simulink library "sm_wheel_loader_lib"  (R2025a)
settings: Solver=VariableStepAuto  StartTime=0.0  StopTime=10.0  RelTol=1e-3
undefined symbols (not defined in the file): AToTOrificeVector, BiPOrificeVector, boomHEArea, boomREArea, BToTOrificeVector, fluids, GRake, GToothL, GToothR, HMPST, HydFcnParams, logLoad, Position, PToAOrificeVector, PToBOrificeVector, RakeL, RakeR, testInput, Wheel_Loader, X, Y, Z
libraries: sm_lib x694, fl_lib x183, nesl_utility x74, SimscapeFluids_lib x62, sdl_lib x25, cvt_components_lib x25, simulink_extras x5, $bdroot x4, wheel_loader_contact_lib x4, ee_lib x2, SignalEditorBlockLib x1, batteryecm_lib x1
(part 15 of 26)

== system sm_wheel_loader_lib/Wheel Loader Vehicle/Actuators/Hydraulic/Valves Linkage/Orifices Lift ==
  Orifice BiP : SimscapeFluids_lib/Isothermal Liquid/Valves & Orifices/Orifices/Orifice (IL)  orifice_type=foundation.enum.constant_variable.variable  constant_orifice_spec=fluids.isothermal_liquid.valves_orifices.orifices.enum.constant_orifice_spec.area  variable_orifice_spec=fluids.isothermal_liquid.valves_orifices.orifices.enum.orifice_spec.table1D_area_opening  orifice_area_constant=1e-3 m^2  p_diff_TLU_constant=[-4, -3, -2, -1, -.5, 0, .5, 1, 2, 3, 4] MPa  vol_flow_TLU_constant=[-2.44, -2.12, -1.68, -1.22, -.84, 0, .85, 1.21, 1.7, 2.09, 2.41] .* 1e-3 m^3/s  S_min=1e-10 m  del_S=0.005 m  open_orientation=fluids.isothermal_liquid.valves_orifices.orifices.enum.orifice_orientation.positive  area_max=0.5e-4 m^2  area_leak=1e-12 m^2  S_TLU=valveData.spoolPosVector mm  orifice_area_TLU=valveData.BiPOrificeAreaVector mm^2  area=inf m^2  Cd=0.7  Re_c=150  smoothing_factor=0  pressure_recovery=simscape.enum.onoff.off  S_vol_flow_TLU=BiPOrificeVector - 1000*(0) mm  p_diff_TLU=[-10000000, -5000000, -2000000, 2000000, 5000000, 10000000] Pa  vol_flow_TLU=[-1e-07, -7.0711e-08, -4.4721e-08, 4.4721e-08, 7.0711e-08, 1e-07; -2.0352e-05, -1.4391e-05, -9.1017e-06, 9.1017e-06, 1.4391e-05, 2.0352e-05; -.0040736, -.0028805, -.0018218, .0018218, .0028805, .0040736; -.011438, -.0080879, -.0051152, .0051152, .0080879, .011438; -.034356, -.024293, -.015364, .015364, .024293, .034356] m^3/s
      settings: InternalSimscapePortConfiguration="{\"Bottom\":[],\"Left\":[{\"id\":\"A\",\"label\":\"A\",\"type\":\"foundation.isothermal_liquid.isothermal_liquid\"},{\"id\":\"S\",\"label\":\"S\",\"type\":\"input\"}],\"Right\":[{\"id\":\"B\",\"label\":\"B\",\"type\":\"foundation.isothermal_liquid.isothermal_liquid\"}],\"Top\":[]}"
  Orifice AT : SimscapeFluids_lib/Isothermal Liquid/Valves & Orifices/Orifices/Orifice (IL)  orifice_type=foundation.enum.constant_variable.variable  constant_orifice_spec=fluids.isothermal_liquid.valves_orifices.orifices.enum.constant_orifice_spec.area  variable_orifice_spec=fluids.isothermal_liquid.valves_orifices.orifices.enum.orifice_spec.table1D_area_opening  orifice_area_constant=1e-3 m^2  p_diff_TLU_constant=[-4, -3, -2, -1, -.5, 0, .5, 1, 2, 3, 4] MPa  vol_flow_TLU_constant=[-2.44, -2.12, -1.68, -1.22, -.84, 0, .85, 1.21, 1.7, 2.09, 2.41] .* 1e-3 m^3/s  S_min=1e-10 m  del_S=0.005 m  open_orientation=fluids.isothermal_liquid.valves_orifices.orifices.enum.orifice_orientation.positive  area_max=0.5e-4 m^2  area_leak=1e-12 m^2  S_TLU=valveData.spoolPosVector mm  orifice_area_TLU=valveData.AtoTOrificeAreaVector mm^2  area=inf m^2  Cd=0.7  Re_c=150  smoothing_factor=0  pressure_recovery=simscape.enum.onoff.off  S_vol_flow_TLU=AToTOrificeVector - 1000*(0) mm  p_diff_TLU=[-10000000, -5000000, -2000000, 2000000, 5000000, 10000000] Pa  vol_flow_TLU=[-1e-07, -7.0711e-08, -4.4721e-08, 4.4721e-08, 7.0711e-08, 1e-07; -2.0352e-05, -1.4391e-05, -9.1017e-06, 9.1017e-06, 1.4391e-05, 2.0352e-05; -.0040736, -.0028805, -.0018218, .0018218, .0028805, .0040736; -.011438, -.0080879, -.0051152, .0051152, .0080879, .011438; -.034356, -.024293, -.015364, .015364, .024293, .034356] m^3/s
      settings: InternalSimscapePortConfiguration="{\"Bottom\":[],\"Left\":[{\"id\":\"A\",\"label\":\"A\",\"type\":\"foundation.isothermal_liquid.isothermal_liquid\"},{\"id\":\"S\",\"label\":\"S\",\"type\":\"input\"}],\"Right\":[{\"id\":\"B\",\"label\":\"B\",\"type\":\"foundation.isothermal_liquid.isothermal_liquid\"}],\"Top\":[]}"
  Orifice BT : SimscapeFluids_lib/Isothermal Liquid/Valves & Orifices/Orifices/Orifice (IL)  orifice_type=foundation.enum.constant_variable.variable  constant_orifice_spec=fluids.isothermal_liquid.valves_orifices.orifices.enum.constant_orifice_spec.area  variable_orifice_spec=fluids.isothermal_liquid.valves_orifices.orifices.enum.orifice_spec.table1D_area_opening  orifice_area_constant=1e-3 m^2  p_diff_TLU_constant=[-4, -3, -2, -1, -.5, 0, .5, 1, 2, 3, 4] MPa  vol_flow_TLU_constant=[-2.44, -2.12, -1.68, -1.22, -.84, 0, .85, 1.21, 1.7, 2.09, 2.41] .* 1e-3 m^3/s  S_min=1e-10 m  del_S=0.005 m  open_orientation=fluids.isothermal_liquid.valves_orifices.orifices.enum.orifice_orientation.positive  area_max=0.5e-4 m^2  area_leak=1e-12 m^2  S_TLU=valveData.spoolPosVector mm  orifice_area_TLU=valveData.BtoTOrificeAreaVector mm^2  area=inf m^2  Cd=0.7  Re_c=150  smoothing_factor=0  pressure_recovery=simscape.enum.onoff.off  S_vol_flow_TLU=BToTOrificeVector - 1000*(0) mm  p_diff_TLU=[-10000000, -5000000, -2000000, 2000000, 5000000, 10000000] Pa  vol_flow_TLU=[-1e-07, -7.0711e-08, -4.4721e-08, 4.4721e-08, 7.0711e-08, 1e-07; -2.0352e-05, -1.4391e-05, -9.1017e-06, 9.1017e-06, 1.4391e-05, 2.0352e-05; -.0040736, -.0028805, -.0018218, .0018218, .0028805, .0040736; -.011438, -.0080879, -.0051152, .0051152, .0080879, .011438; -.034356, -.024293, -.015364, .015364, .024293, .034356] m^3/s
      settings: InternalSimscapePortConfiguration="{\"Bottom\":[],\"Left\":[{\"id\":\"A\",\"label\":\"A\",\"type\":\"foundation.isothermal_liquid.isothermal_liquid\"},{\"id\":\"S\",\"label\":\"S\",\"type\":\"input\"}],\"Right\":[{\"id\":\"B\",\"label\":\"B\",\"type\":\"foundation.isothermal_liquid.isothermal_liquid\"}],\"Top\":[]}"
  Orifice PA : SimscapeFluids_lib/Isothermal Liquid/Valves & Orifices/Orifices/Orifice (IL)  orifice_type=foundation.enum.constant_variable.variable  constant_orifice_spec=fluids.isothermal_liquid.valves_orifices.orifices.enum.constant_orifice_spec.area  variable_orifice_spec=fluids.isothermal_liquid.valves_orifices.orifices.enum.orifice_spec.table1D_area_opening  orifice_area_constant=1e-3 m^2  p_diff_TLU_constant=[-4, -3, -2, -1, -.5, 0, .5, 1, 2, 3, 4] MPa  vol_flow_TLU_constant=[-2.44, -2.12, -1.68, -1.22, -.84, 0, .85, 1.21, 1.7, 2.09, 2.41] .* 1e-3 m^3/s  S_min=1e-10 m  del_S=0.005 m  open_orientation=fluids.isothermal_liquid.valves_orifices.orifices.enum.orifice_orientation.positive  area_max=0.5e-4 m^2  area_leak=1e-12 m^2  S_TLU=valveData.spoolPosVector mm  orifice_area_TLU=valveData.PtoAOrificeAreaVector mm^2  area=inf m^2  Cd=0.7  Re_c=150  smoothing_factor=0  pressure_recovery=simscape.enum.onoff.off  S_vol_flow_TLU=PToAOrificeVector - 1000*(0) mm  p_diff_TLU=[-10000000, -5000000, -2000000, 2000000, 5000000, 10000000] Pa  vol_flow_TLU=[-1e-07, -7.0711e-08, -4.4721e-08, 4.4721e-08, 7.0711e-08, 1e-07; -2.0352e-05, -1.4391e-05, -9.1017e-06, 9.1017e-06, 1.4391e-05, 2.0352e-05; -.0040736, -.0028805, -.0018218, .0018218, .0028805, .0040736; -.011438, -.0080879, -.0051152, .0051152, .0080879, .011438; -.034356, -.024293, -.015364, .015364, .024293, .034356] m^3/s
      settings: InternalSimscapePortConfiguration="{\"Bottom\":[],\"Left\":[{\"id\":\"A\",\"label\":\"A\",\"type\":\"foundation.isothermal_liquid.isothermal_liquid\"},{\"id\":\"S\",\"label\":\"S\",\"type\":\"input\"}],\"Right\":[{\"id\":\"B\",\"label\":\"B\",\"type\":\"foundation.isothermal_liquid.isothermal_liquid\"}],\"Top\":[]}"
  Orifice PB : SimscapeFluids_lib/Isothermal Liquid/Valves & Orifices/Orifices/Orifice (IL)  orifice_type=foundation.enum.constant_variable.variable  constant_orifice_spec=fluids.isothermal_liquid.valves_orifices.orifices.enum.constant_orifice_spec.area  variable_orifice_spec=fluids.isothermal_liquid.valves_orifices.orifices.enum.orifice_spec.table1D_area_opening  orifice_area_constant=1e-3 m^2  p_diff_TLU_constant=[-4, -3, -2, -1, -.5, 0, .5, 1, 2, 3, 4] MPa  vol_flow_TLU_constant=[-2.44, -2.12, -1.68, -1.22, -.84, 0, .85, 1.21, 1.7, 2.09, 2.41] .* 1e-3 m^3/s  S_min=1e-10 m  del_S=0.005 m  open_orientation=fluids.isothermal_liquid.valves_orifices.orifices.enum.orifice_orientation.positive  area_max=0.5e-4 m^2  area_leak=1e-12 m^2  S_TLU=valveData.spoolPosVector mm  orifice_area_TLU=valveData.PtoBOrificeAreaVector mm^2  area=inf m^2  Cd=0.7  Re_c=150  smoothing_factor=0  pressure_recovery=simscape.enum.onoff.off  S_vol_flow_TLU=PToBOrificeVector - 1000*(0) mm  p_diff_TLU=[-10000000, -5000000, -2000000, 2000000, 5000000, 10000000] Pa  vol_flow_TLU=[-1e-07, -7.0711e-08, -4.4721e-08, 4.4721e-08, 7.0711e-08, 1e-07; -2.0352e-05, -1.4391e-05, -9.1017e-06, 9.1017e-06, 1.4391e-05, 2.0352e-05; -.0040736, -.0028805, -.0018218, .0018218, .0028805, .0040736; -.011438, -.0080879, -.0051152, .0051152, .0080879, .011438; -.034356, -.024293, -.015364, .015364, .024293, .034356] m^3/s
      settings: InternalSimscapePortConfiguration="{\"Bottom\":[],\"Left\":[{\"id\":\"A\",\"label\":\"A\",\"type\":\"foundation.isothermal_liquid.isothermal_liquid\"},{\"id\":\"S\",\"label\":\"S\",\"type\":\"input\"}],\"Right\":[{\"id\":\"B\",\"label\":\"B\",\"type\":\"foundation.isothermal_liquid.isothermal_liquid\"}],\"Top\":[]}"
  PS Abs : fl_lib/Physical Signals/Nonlinear Operators/PS Abs  ZeroCross=true
      settings: InternalSimscapePortConfiguration="{\"Bottom\":[],\"Left\":[{\"id\":\"I\",\"label\":\"\",\"type\":\"input\"}],\"Right\":[{\"id\":\"O\",\"label\":\"\",\"type\":\"output\"}],\"Top\":[]}"
  PS Gain : fl_lib/Physical Signals/Functions/PS Gain  gain=-1
  PS Gain1 : fl_lib/Physical Signals/Functions/PS Gain  gain=-1
  S : PMIOPort  Side=Left
  P : PMIOPort  Port=2  Side=Left
  T : PMIOPort  Port=3  Side=Left
  BiPIn : PMIOPort  Port=4  Side=Left
  A : PMIOPort  Port=5  Side=Right
  B : PMIOPort  Port=6  Side=Right
  BiPOut : PMIOPort  Port=7  Side=Right
  connections:
  Orifice BT/LConn2 -- PS Gain1/RConn1
  Orifice PA/LConn2 -- PS Gain/RConn1
  PS Gain1/LConn1 -- Orifice AT/LConn2 -- S/RConn1 -- PS Abs/LConn1 -- Orifice PB/LConn2 -- PS Gain/LConn1
  Orifice BT/RConn1 -- Orifice AT/RConn1 -- T/RConn1
  Orifice BiP/RConn1 -- BiPOut/RConn1
  Orifice BiP/LConn1 -- BiPIn/RConn1
  Orifice PA/RConn1 -- A/RConn1 -- Orifice AT/LConn1
  Orifice PA/LConn1 -- P/RConn1 -- Orifice PB/LConn1
  Orifice PB/RConn1 -- B/RConn1 -- Orifice BT/LConn1
  PS Abs/RConn1 -- Orifice BiP/LConn2

== system sm_wheel_loader_lib/Wheel Loader Vehicle/Actuators/Hydraulic/Valves Linkage/Orifices Tilt ==
  Orifice BiP : SimscapeFluids_lib/Isothermal Liquid/Valves & Orifices/Orifices/Orifice (IL)  orifice_type=foundation.enum.constant_variable.variable  constant_orifice_spec=fluids.isothermal_liquid.valves_orifices.orifices.enum.constant_orifice_spec.area  variable_orifice_spec=fluids.isothermal_liquid.valves_orifices.orifices.enum.orifice_spec.table1D_area_opening  orifice_area_constant=1e-3 m^2  p_diff_TLU_constant=[-4, -3, -2, -1, -.5, 0, .5, 1, 2, 3, 4] MPa  vol_flow_TLU_constant=[-2.44, -2.12, -1.68, -1.22, -.84, 0, .85, 1.21, 1.7, 2.09, 2.41] .* 1e-3 m^3/s  S_min=1e-10 m  del_S=0.005 m  open_orientation=fluids.isothermal_liquid.valves_orifices.orifices.enum.orifice_orientation.positive  area_max=0.5e-4 m^2  area_leak=1e-12 m^2  S_TLU=valveData.spoolPosVector mm  orifice_area_TLU=valveData.BiPOrificeAreaVector mm^2  area=inf m^2  Cd=0.7  Re_c=150  smoothing_factor=0  pressure_recovery=simscape.enum.onoff.off  S_vol_flow_TLU=BiPOrificeVector - 1000*(0) mm  p_diff_TLU=[-10000000, -5000000, -2000000, 2000000, 5000000, 10000000] Pa  vol_flow_TLU=[-1e-07, -7.0711e-08, -4.4721e-08, 4.4721e-08, 7.0711e-08, 1e-07; -2.0352e-05, -1.4391e-05, -9.1017e-06, 9.1017e-06, 1.4391e-05, 2.0352e-05; -.0040736, -.0028805, -.0018218, .0018218, .0028805, .0040736; -.011438, -.0080879, -.0051152, .0051152, .0080879, .011438; -.034356, -.024293, -.015364, .015364, .024293, .034356] m^3/s
      settings: InternalSimscapePortConfiguration="{\"Bottom\":[],\"Left\":[{\"id\":\"A\",\"label\":\"A\",\"type\":\"foundation.isothermal_liquid.isothermal_liquid\"},{\"id\":\"S\",\"label\":\"S\",\"type\":\"input\"}],\"Right\":[{\"id\":\"B\",\"label\":\"B\",\"type\":\"foundation.isothermal_liquid.isothermal_liquid\"}],\"Top\":[]}"
  Orifice AT : SimscapeFluids_lib/Isothermal Liquid/Valves & Orifices/Orifices/Orifice (IL)  orifice_type=foundation.enum.constant_variable.variable  constant_orifice_spec=fluids.isothermal_liquid.valves_orifices.orifices.enum.constant_orifice_spec.area  variable_orifice_spec=fluids.isothermal_liquid.valves_orifices.orifices.enum.orifice_spec.table1D_area_opening  orifice_area_constant=1e-3 m^2  p_diff_TLU_constant=[-4, -3, -2, -1, -.5, 0, .5, 1, 2, 3, 4] MPa  vol_flow_TLU_constant=[-2.44, -2.12, -1.68, -1.22, -.84, 0, .85, 1.21, 1.7, 2.09, 2.41] .* 1e-3 m^3/s  S_min=1e-10 m  del_S=0.005 m  open_orientation=fluids.isothermal_liquid.valves_orifices.orifices.enum.orifice_orientation.positive  area_max=0.5e-4 m^2  area_leak=1e-12 m^2  S_TLU=valveData.spoolPosVector mm  orifice_area_TLU=valveData.AtoTOrificeAreaVector mm^2  area=inf m^2  Cd=0.7  Re_c=150  smoothing_factor=0  pressure_recovery=simscape.enum.onoff.off  S_vol_flow_TLU=AToTOrificeVector - 1000*(0) mm  p_diff_TLU=[-10000000, -5000000, -2000000, 2000000, 5000000, 10000000] Pa  vol_flow_TLU=[-1e-07, -7.0711e-08, -4.4721e-08, 4.4721e-08, 7.0711e-08, 1e-07; -2.0352e-05, -1.4391e-05, -9.1017e-06, 9.1017e-06, 1.4391e-05, 2.0352e-05; -.0040736, -.0028805, -.0018218, .0018218, .0028805, .0040736; -.011438, -.0080879, -.0051152, .0051152, .0080879, .011438; -.034356, -.024293, -.015364, .015364, .024293, .034356] m^3/s
      settings: InternalSimscapePortConfiguration="{\"Bottom\":[],\"Left\":[{\"id\":\"A\",\"label\":\"A\",\"type\":\"foundation.isothermal_liquid.isothermal_liquid\"},{\"id\":\"S\",\"label\":\"S\",\"type\":\"input\"}],\"Right\":[{\"id\":\"B\",\"label\":\"B\",\"type\":\"foundation.isothermal_liquid.isothermal_liquid\"}],\"Top\":[]}"
  Orifice BT : SimscapeFluids_lib/Isothermal Liquid/Valves & Orifices/Orifices/Orifice (IL)  orifice_type=foundation.enum.constant_variable.variable  constant_orifice_spec=fluids.isothermal_liquid.valves_orifices.orifices.enum.constant_orifice_spec.area  variable_orifice_spec=fluids.isothermal_liquid.valves_orifices.orifices.enum.orifice_spec.table1D_area_opening  orifice_area_constant=1e-3 m^2  p_diff_TLU_constant=[-4, -3, -2, -1, -.5, 0, .5, 1, 2, 3, 4] MPa  vol_flow_TLU_constant=[-2.44, -2.12, -1.68, -1.22, -.84, 0, .85, 1.21, 1.7, 2.09, 2.41] .* 1e-3 m^3/s  S_min=1e-10 m  del_S=0.005 m  open_orientation=fluids.isothermal_liquid.valves_orifices.orifices.enum.orifice_orientation.positive  area_max=0.5e-4 m^2  area_leak=1e-12 m^2  S_TLU=valveData.spoolPosVector mm  orifice_area_TLU=valveData.BtoTOrificeAreaVector mm^2  area=inf m^2  Cd=0.7  Re_c=150  smoothing_factor=0  pressure_recovery=simscape.enum.onoff.off  S_vol_flow_TLU=BToTOrificeVector - 1000*(0) mm  p_diff_TLU=[-10000000, -5000000, -2000000, 2000000, 5000000, 10000000] Pa  vol_flow_TLU=[-1e-07, -7.0711e-08, -4.4721e-08, 4.4721e-08, 7.0711e-08, 1e-07; -2.0352e-05, -1.4391e-05, -9.1017e-06, 9.1017e-06, 1.4391e-05, 2.0352e-05; -.0040736, -.0028805, -.0018218, .0018218, .0028805, .0040736; -.011438, -.0080879, -.0051152, .0051152, .0080879, .011438; -.034356, -.024293, -.015364, .015364, .024293, .034356] m^3/s
      settings: InternalSimscapePortConfiguration="{\"Bottom\":[],\"Left\":[{\"id\":\"A\",\"label\":\"A\",\"type\":\"foundation.isothermal_liquid.isothermal_liquid\"},{\"id\":\"S\",\"label\":\"S\",\"type\":\"input\"}],\"Right\":[{\"id\":\"B\",\"label\":\"B\",\"type\":\"foundation.isothermal_liquid.isothermal_liquid\"}],\"Top\":[]}"
  Orifice PA : SimscapeFluids_lib/Isothermal Liquid/Valves & Orifices/Orifices/Orifice (IL)  orifice_type=foundation.enum.constant_variable.variable  constant_orifice_spec=fluids.isothermal_liquid.valves_orifices.orifices.enum.constant_orifice_spec.area  variable_orifice_spec=fluids.isothermal_liquid.valves_orifices.orifices.enum.orifice_spec.table1D_area_opening  orifice_area_constant=1e-3 m^2  p_diff_TLU_constant=[-4, -3, -2, -1, -.5, 0, .5, 1, 2, 3, 4] MPa  vol_flow_TLU_constant=[-2.44, -2.12, -1.68, -1.22, -.84, 0, .85, 1.21, 1.7, 2.09, 2.41] .* 1e-3 m^3/s  S_min=1e-10 m  del_S=0.005 m  open_orientation=fluids.isothermal_liquid.valves_orifices.orifices.enum.orifice_orientation.positive  area_max=0.5e-4 m^2  area_leak=1e-12 m^2  S_TLU=valveData.spoolPosVector mm  orifice_area_TLU=valveData.PtoAOrificeAreaVector mm^2  area=inf m^2  Cd=0.7  Re_c=150  smoothing_factor=0  pressure_recovery=simscape.enum.onoff.off  S_vol_flow_TLU=PToAOrificeVector - 1000*(0) mm  p_diff_TLU=[-10000000, -5000000, -2000000, 2000000, 5000000, 10000000] Pa  vol_flow_TLU=[-1e-07, -7.0711e-08, -4.4721e-08, 4.4721e-08, 7.0711e-08, 1e-07; -2.0352e-05, -1.4391e-05, -9.1017e-06, 9.1017e-06, 1.4391e-05, 2.0352e-05; -.0040736, -.0028805, -.0018218, .0018218, .0028805, .0040736; -.011438, -.0080879, -.0051152, .0051152, .0080879, .011438; -.034356, -.024293, -.015364, .015364, .024293, .034356] m^3/s
      settings: InternalSimscapePortConfiguration="{\"Bottom\":[],\"Left\":[{\"id\":\"A\",\"label\":\"A\",\"type\":\"foundation.isothermal_liquid.isothermal_liquid\"},{\"id\":\"S\",\"label\":\"S\",\"type\":\"input\"}],\"Right\":[{\"id\":\"B\",\"label\":\"B\",\"type\":\"foundation.isothermal_liquid.isothermal_liquid\"}],\"Top\":[]}"
  Orifice PB : SimscapeFluids_lib/Isothermal Liquid/Valves & Orifices/Orifices/Orifice (IL)  orifice_type=foundation.enum.constant_variable.variable  constant_orifice_spec=fluids.isothermal_liquid.valves_orifices.orifices.enum.constant_orifice_spec.area  variable_orifice_spec=fluids.isothermal_liquid.valves_orifices.orifices.enum.orifice_spec.table1D_area_opening  orifice_area_constant=1e-3 m^2  p_diff_TLU_constant=[-4, -3, -2, -1, -.5, 0, .5, 1, 2, 3, 4] MPa  vol_flow_TLU_constant=[-2.44, -2.12, -1.68, -1.22, -.84, 0, .85, 1.21, 1.7, 2.09, 2.41] .* 1e-3 m^3/s  S_min=1e-10 m  del_S=0.005 m  open_orientation=fluids.isothermal_liquid.valves_orifices.orifices.enum.orifice_orientation.positive  area_max=0.5e-4 m^2  area_leak=1e-12 m^2  S_TLU=valveData.spoolPosVector mm  orifice_area_TLU=valveData.PtoBOrificeAreaVector mm^2  area=inf m^2  Cd=0.7  Re_c=150  smoothing_factor=0  pressure_recovery=simscape.enum.onoff.off  S_vol_flow_TLU=PToBOrificeVector - 1000*(0) mm  p_diff_TLU=[-10000000, -5000000, -2000000, 2000000, 5000000, 10000000] Pa  vol_flow_TLU=[-1e-07, -7.0711e-08, -4.4721e-08, 4.4721e-08, 7.0711e-08, 1e-07; -2.0352e-05, -1.4391e-05, -9.1017e-06, 9.1017e-06, 1.4391e-05, 2.0352e-05; -.0040736, -.0028805, -.0018218, .0018218, .0028805, .0040736; -.011438, -.0080879, -.0051152, .0051152, .0080879, .011438; -.034356, -.024293, -.015364, .015364, .024293, .034356] m^3/s
      settings: InternalSimscapePortConfiguration="{\"Bottom\":[],\"Left\":[{\"id\":\"A\",\"label\":\"A\",\"type\":\"foundation.isothermal_liquid.isothermal_liquid\"},{\"id\":\"S\",\"label\":\"S\",\"type\":\"input\"}],\"Right\":[{\"id\":\"B\",\"label\":\"B\",\"type\":\"foundation.isothermal_liquid.isothermal_liquid\"}],\"Top\":[]}"
  PS Abs : fl_lib/Physical Signals/Nonlinear Operators/PS Abs  ZeroCross=true
      settings: InternalSimscapePortConfiguration="{\"Bottom\":[],\"Left\":[{\"id\":\"I\",\"label\":\"\",\"type\":\"input\"}],\"Right\":[{\"id\":\"O\",\"label\":\"\",\"type\":\"output\"}],\"Top\":[]}"
  PS Gain : fl_lib/Physical Signals/Functions/PS Gain  gain=-1
  PS Gain1 : fl_lib/Physical Signals/Functions/PS Gain  gain=-1
  S : PMIOPort  Side=Left
  P : PMIOPort  Port=2  Side=Left
  T : PMIOPort  Port=3  Side=Left
  BiPIn : PMIOPort  Port=4  Side=Left
  A : PMIOPort  Port=5  Side=Right
  B : PMIOPort  Port=6  Side=Right
  BiPOut : PMIOPort  Port=7  Side=Right
  connections:
  Orifice BT/LConn2 -- PS Gain1/RConn1
  Orifice PA/LConn2 -- PS Gain/RConn1
  PS Abs/LConn1 -- S/RConn1 -- PS Gain/LConn1 -- Orifice PB/LConn2 -- Orifice AT/LConn2 -- PS Gain1/LConn1
  T/RConn1 -- Orifice AT/RConn1 -- Orifice BT/RConn1
  Orifice BiP/RConn1 -- BiPOut/RConn1
  Orifice BiP/LConn1 -- BiPIn/RConn1
  Orifice PA/RConn1 -- A/RConn1 -- Orifice AT/LConn1
  Orifice PA/LConn1 -- P/RConn1 -- Orifice PB/LConn1
  Orifice BT/LConn1 -- Orifice PB/RConn1 -- B/RConn1
  PS Abs/RConn1 -- Orifice BiP/LConn2

== system sm_wheel_loader_lib/Wheel Loader Vehicle/Actuators/Ideal/Power Draw/Limit w ==
  PS Abs : fl_lib/Physical Signals/Nonlinear Operators/PS Abs  ZeroCross=true
      settings: InternalSimscapePortConfiguration="{\"Bottom\":[],\"Left\":[{\"id\":\"I\",\"label\":\"\",\"type\":\"input\"}],\"Right\":[{\"id\":\"O\",\"label\":\"\",\"type\":\"output\"}],\"Top\":[]}"
  PS Constant : fl_lib/Physical Signals/Sources/PS Constant  constant=1e-3 rad/s
  PS Max : fl_lib/Physical Signals/Nonlinear Operators/PS Max  ZeroCross=true
      settings: InternalSimscapePortConfiguration="{\"Bottom\":[],\"Left\":[{\"id\":\"I1\",\"label\":\"\",\"type\":\"input\"},{\"id\":\"I2\",\"label\":\"\",\"type\":\"input\"}],\"Right\":[{\"id\":\"O\",\"label\":\"\",\"type\":\"output\"}],\"Top\":[]}"
  PS Product : fl_lib/Physical Signals/Functions/PS Product
  PS Sign : fl_lib/Physical Signals/Nonlinear Operators/PS Sign
      settings: InternalSimscapePortConfiguration="{\"Bottom\":[],\"Left\":[{\"id\":\"I\",\"label\":\"\",\"type\":\"input\"}],\"Right\":[{\"id\":\"O\",\"label\":\"\",\"type\":\"output\"}],\"Top\":[]}"
  wLim : PMIOPort  Side=Right
  w : PMIOPort  Port=2  Side=Left
  connections:
  wLim/RConn1 -- PS Product/RConn1
  PS Max/LConn1 -- PS Abs/RConn1
  PS Max/LConn2 -- PS Constant/RConn1
  PS Product/LConn2 -- PS Max/RConn1
  w/RConn1 -- PS Sign/LConn1 -- PS Abs/LConn1
  PS Product/LConn1 -- PS Sign/RConn1

== system sm_wheel_loader_lib/Wheel Loader Vehicle/Driveline/Driveline/Driveline 1D/Driveline ==
  Damper : fl_lib/Mechanical/Rotational Elements/Rotational Damper  D=HMPST.DriveshaftF.D N*m*s/rad  w_specify=off  w_priority=None  w=0 rad/s  w_nominal_specify=off  w_nominal_value=1  w_nominal_unit=rad/s  t_specify=off  t_priority=None  t=0 N*m  t_nominal_specify=off  t_nominal_value=1  t_nominal_unit=N*m
  Differential Front : sdl_lib/Gears/Differential  driveshaft_location=2  cd_ratio=HMPST.Differential.Ratio  friction_model=2  efficiency=[ 0.99 0.99 ]  temperature_TLU=[ 280 300 320 ] K  efficiency_ss_TLU=[ 0.95 0.9 0.85 ]  efficiency_cd_TLU=[ 0.95 0.9 0.85 ]  pwr_thr=[ 0.001 0.001 ] W  mu_visc=[0 0] N*m/(rad/s)  model_inertia=1  sun_inertia=1e-10 kg*m^2  sun_radius=0.01 m  carrier_inertia=0.1 kg*m^2  planet_inertia=0.1 kg*m^2  planet_mass=1e-10 kg  thermal_mass=50 J/K  T_init=300 K
  Differential Rear : sdl_lib/Gears/Differential  driveshaft_location=2  cd_ratio=HMPST.Differential.Ratio  friction_model=sdl.enum.gear_friction.none  efficiency=[ 0.99 0.99 ]  temperature_TLU=[ 280 300 320 ] K  efficiency_ss_TLU=[ 0.95 0.9 0.85 ]  efficiency_cd_TLU=[ 0.95 0.9 0.85 ]  pwr_thr=[ 0.001 0.001 ] W  mu_visc=[ 0 0 ] N*m/(rad/s)  model_inertia=1  sun_inertia=1e-10 kg*m^2  sun_radius=0.01 m  carrier_inertia=0.1 kg*m^2  planet_inertia=0.1 kg*m^2  planet_mass=1e-10 kg  thermal_mass=50 J/K  T_init=300 K
  Gear Output Transfer : sdl_lib/Gears/Simple Gear  ratio=HMPST.OutputTransferGearPair.Ratio  rotation_direction=sdl.enum.shaftOutputDirection.opposite  friction_model=sdl.enum.gear_efficiencies_load.off  T_noload=0.1 N*m  T_nom=5 N*m  efficiency_nom=0.8  efficiency=0.99  temperature_TLU=[ 280 300 320 ] K  load_TLU=[ 1 5 10 ] N*m  efficiency_TLU=[ 0.995 0.95 0.91 ]  efficiency_TLU2=[ 0.85 0.8 0.75; 0.95 0.9 0.85; 0.85 0.8 0.7 ]  w_thr=0.01 rad/s  pwr_thr=0.001 W  enable_backlash=false  hardstop_model=simscape.enum.hardstop.smooth  backlash_distance=1e-3 mm  r_base=0.1 m  transition=1e-4 mm  backlash_stiffness=1e6 N/m  backlash_damping=1e3 N*s/m  coeff_rest=0.7  v_tol=0.001 m/s  f_tol=0 N  mu_visc=[ 0 0] N*m/(rad/s)  thermal_mass=1000 J/K  temperature_specify=off  temperature_priority=High  temperature=300 K  temperature_nominal_specify=off  temperature_nominal_value=1  temperature_nominal_unit=K  x_backlash_specify=off  x_backlash_priority=None  x_backlash=0 mm  x_backlash_nominal_specify=off  x_backlash_nominal_value=1  x_backlash_nominal_unit=mm  f_hardstop_specify=off  f_hardstop_priority=None  f_hardstop=0 N  f_hardstop_nominal_specify=off  f_hardstop_nominal_value=1  f_hardstop_nominal_unit=N  v_backlash_specify=off  v_backlash_priority=None  v_backlash=0 m/s  v_backlash_nominal_specify=off  v_backlash_nominal_value=1  v_backlash_nominal_unit=m/s
  Gear Sun FR : sdl_lib/Gears/Simple Gear  ratio=HMPST.FinalDrive.Ratio  rotation_direction=sdl.enum.shaftOutputDirection.opposite  friction_model=2  T_noload=0.1 N*m  T_nom=5 N*m  efficiency_nom=0.8  efficiency=0.99  temperature_TLU=[ 280 300 320 ] K  load_TLU=[ 1 5 10 ] N*m  efficiency_TLU=[ 0.995 0.95 0.91 ]  efficiency_TLU2=[ 0.85 0.8 0.75; 0.95 0.9 0.85; 0.85 0.8 0.7 ]  w_thr=0.01 rad/s  pwr_thr=0.001 W  enable_backlash=false  hardstop_model=simscape.enum.hardstop.smooth  backlash_distance=1e-3 mm  r_base=0.1 m  transition=1e-4 mm  backlash_stiffness=1e6 N/m  backlash_damping=1e3 N*s/m  coeff_rest=0.7  v_tol=0.001 m/s  f_tol=0 N  mu_visc=[0 0] N*m/(rad/s)  thermal_mass=1000 J/K  temperature_specify=off  temperature_priority=High  temperature=300 K  temperature_nominal_specify=off  temperature_nominal_value=1  temperature_nominal_unit=K  x_backlash_specify=off  x_backlash_priority=None  x_backlash=0 mm  x_backlash_nominal_specify=off  x_backlash_nominal_value=1  x_backlash_nominal_unit=mm  f_hardstop_specify=off  f_hardstop_priority=None  f_hardstop=0 N  f_hardstop_nominal_specify=off  f_hardstop_nominal_value=1  f_hardstop_nominal_unit=N  v_backlash_specify=off  v_backlash_priority=None  v_backlash=0 m/s  v_backlash_nominal_specify=off  v_backlash_nominal_value=1  v_backlash_nominal_unit=m/s
  Gear Sun LF : sdl_lib/Gears/Simple Gear  ratio=HMPST.FinalDrive.Ratio  rotation_direction=sdl.enum.shaftOutputDirection.opposite  friction_model=2  T_noload=0.1 N*m  T_nom=5 N*m  efficiency_nom=0.8  efficiency=0.99  temperature_TLU=[ 280 300 320 ] K  load_TLU=[ 1 5 10 ] N*m  efficiency_TLU=[ 0.995 0.95 0.91 ]  efficiency_TLU2=[ 0.85 0.8 0.75; 0.95 0.9 0.85; 0.85 0.8 0.7 ]  w_thr=0.01 rad/s  pwr_thr=0.001 W  enable_backlash=false  hardstop_model=simscape.enum.hardstop.smooth  backlash_distance=1e-3 mm  r_base=0.1 m  transition=1e-4 mm  backlash_stiffness=1e6 N/m  backlash_damping=1e3 N*s/m  coeff_rest=0.7  v_tol=0.001 m/s  f_tol=0 N  mu_visc=[0 0] N*m/(rad/s)  thermal_mass=1000 J/K  temperature_specify=off  temperature_priority=High  temperature=300 K  temperature_nominal_specify=off  temperature_nominal_value=1  temperature_nominal_unit=K  x_backlash_specify=off  x_backlash_priority=None  x_backlash=0 mm  x_backlash_nominal_specify=off  x_backlash_nominal_value=1  x_backlash_nominal_unit=mm  f_hardstop_specify=off  f_hardstop_priority=None  f_hardstop=0 N  f_hardstop_nominal_specify=off  f_hardstop_nominal_value=1  f_hardstop_nominal_unit=N  v_backlash_specify=off  v_backlash_priority=None  v_backlash=0 m/s  v_backlash_nominal_specify=off  v_backlash_nominal_value=1  v_backlash_nominal_unit=m/s
  Gear Sun LR : sdl_lib/Gears/Simple Gear  ratio=HMPST.FinalDrive.Ratio  rotation_direction=sdl.enum.shaftOutputDirection.opposite  friction_model=sdl.enum.gear_efficiencies_load.off  T_noload=0.1 N*m  T_nom=5 N*m  efficiency_nom=0.8  efficiency=0.99  temperature_TLU=[ 280 300 320 ] K  load_TLU=[ 1 5 10 ] N*m  efficiency_TLU=[ 0.995 0.95 0.91 ]  efficiency_TLU2=[ 0.85 0.8 0.75; 0.95 0.9 0.85; 0.85 0.8 0.7 ]  w_thr=0.01 rad/s  pwr_thr=0.001 W  enable_backlash=false  hardstop_model=simscape.enum.hardstop.smooth  backlash_distance=1e-3 mm  r_base=0.1 m  transition=1e-4 mm  backlash_stiffness=1e6 N/m  backlash_damping=1e3 N*s/m  coeff_rest=0.7  v_tol=0.001 m/s  f_tol=0 N  mu_visc=[ 0 0] N*m/(rad/s)  thermal_mass=1000 J/K  temperature_specify=off  temperature_priority=High  temperature=300 K  temperature_nominal_specify=off  temperature_nominal_value=1  temperature_nominal_unit=K  x_backlash_specify=off  x_backlash_priority=None  x_backlash=0 mm  x_backlash_nominal_specify=off  x_backlash_nominal_value=1  x_backlash_nominal_unit=mm  f_hardstop_specify=off  f_hardstop_priority=None  f_hardstop=0 N  f_hardstop_nominal_specify=off  f_hardstop_nominal_value=1  f_hardstop_nominal_unit=N  v_backlash_specify=off  v_backlash_priority=None  v_backlash=0 m/s  v_backlash_nominal_specify=off  v_backlash_nominal_value=1  v_backlash_nominal_unit=m/s
  Gear Sun RR : sdl_lib/Gears/Simple Gear  ratio=HMPST.FinalDrive.Ratio  rotation_direction=sdl.enum.shaftOutputDirection.opposite  friction_model=sdl.enum.gear_efficiencies_load.off  T_noload=0.1 N*m  T_nom=5 N*m  efficiency_nom=0.8  efficiency=0.99  temperature_TLU=[ 280 300 320 ] K  load_TLU=[ 1 5 10 ] N*m  efficiency_TLU=[ 0.995 0.95 0.91 ]  efficiency_TLU2=[ 0.85 0.8 0.75; 0.95 0.9 0.85; 0.85 0.8 0.7 ]  w_thr=0.01 rad/s  pwr_thr=0.001 W  enable_backlash=false  hardstop_model=simscape.enum.hardstop.smooth  backlash_distance=1e-3 mm  r_base=0.1 m  transition=1e-4 mm  backlash_stiffness=1e6 N/m  backlash_damping=1e3 N*s/m  coeff_rest=0.7  v_tol=0.001 m/s  f_tol=0 N  mu_visc=[ 0 0] N*m/(rad/s)  thermal_mass=1000 J/K  temperature_specify=off  temperature_priority=High  temperature=300 K  temperature_nominal_specify=off  temperature_nominal_value=1  temperature_nominal_unit=K  x_backlash_specify=off  x_backlash_priority=None  x_backlash=0 mm  x_backlash_nominal_specify=off  x_backlash_nominal_value=1  x_backlash_nominal_unit=mm  f_hardstop_specify=off  f_hardstop_priority=None  f_hardstop=0 N  f_hardstop_nominal_specify=off  f_hardstop_nominal_value=1  f_hardstop_nominal_unit=N  v_backlash_specify=off  v_backlash_priority=None  v_backlash=0 m/s  v_backlash_nominal_specify=off  v_backlash_nominal_value=1  v_backlash_nominal_unit=m/s
  Inertia Carrier FL : fl_lib/Mechanical/Rotational Elements/Inertia  inertia=1 kg*m^2  num_ports=foundation.enum.numPorts2.two  w_specify=off  w_priority=High  w=0 rad/s  w_nominal_specify=off  w_nominal_value=1  w_nominal_unit=rad/s  t_specify=off  t_priority=None  t=0 N*m  t_nominal_specify=off  t_nominal_value=1  t_nominal_unit=N*m
      settings: InternalSimscapePortConfiguration="{\"Bottom\":[],\"Left\":[{\"id\":\"I\",\"label\":\"\",\"type\":\"foundation.mechanical.rotational.rotational\"}],\"Right\":[{\"id\":\"J\",\"label\":\"\",\"type\":\"foundation.mechanical.rotational.rotational\"}],\"Top\":[]}"
  Inertia Carrier FR : fl_lib/Mechanical/Rotational Elements/Inertia  inertia=1 kg*m^2  num_ports=foundation.enum.numPorts2.two  w_specify=off  w_priority=High  w=0 rad/s  w_nominal_specify=off  w_nominal_value=1  w_nominal_unit=rad/s  t_specify=off  t_priority=None  t=0 N*m  t_nominal_specify=off  t_nominal_value=1  t_nominal_unit=N*m
      settings: InternalSimscapePortConfiguration="{\"Bottom\":[],\"Left\":[{\"id\":\"I\",\"label\":\"\",\"type\":\"foundation.mechanical.rotational.rotational\"}],\"Right\":[{\"id\":\"J\",\"label\":\"\",\"type\":\"foundation.mechanical.rotational.rotational\"}],\"Top\":[]}"
  Inertia Carrier RL : fl_lib/Mechanical/Rotational Elements/Inertia  inertia=1 kg*m^2  num_ports=foundation.enum.numPorts2.two  w_specify=off  w_priority=High  w=0 rad/s  w_nominal_specify=off  w_nominal_value=1  w_nominal_unit=rad/s  t_specify=off  t_priority=None  t=0 N*m  t_nominal_specify=off  t_nominal_value=1  t_nominal_unit=N*m
      settings: InternalSimscapePortConfiguration="{\"Bottom\":[],\"Left\":[{\"id\":\"I\",\"label\":\"\",\"type\":\"foundation.mechanical.rotational.rotational\"}],\"Right\":[{\"id\":\"J\",\"label\":\"\",\"type\":\"foundation.mechanical.rotational.rotational\"}],\"Top\":[]}"
  Inertia Carrier RR : fl_lib/Mechanical/Rotational Elements/Inertia  inertia=1 kg*m^2  num_ports=foundation.enum.numPorts2.two  w_specify=off  w_priority=High  w=0 rad/s  w_nominal_specify=off  w_nominal_value=1  w_nominal_unit=rad/s  t_specify=off  t_priority=None  t=0 N*m  t_nominal_specify=off  t_nominal_value=1  t_nominal_unit=N*m
      settings: InternalSimscapePortConfiguration="{\"Bottom\":[],\"Left\":[{\"id\":\"I\",\"label\":\"\",\"type\":\"foundation.mechanical.rotational.rotational\"}],\"Right\":[{\"id\":\"J\",\"label\":\"\",\"type\":\"foundation.mechanical.rotational.rotational\"}],\"Top\":[]}"
  Inertia Driveshaft Rear : fl_lib/Mechanical/Rotational Elements/Inertia  inertia=HMPST.DriveshaftR.J kg*m^2  num_ports=foundation.enum.numPorts2.two  w_specify=off  w_priority=High  w=0 rad/s  w_nominal_specify=off  w_nominal_value=1  w_nominal_unit=rad/s  t_specify=off  t_priority=None  t=0 N*m  t_nominal_specify=off  t_nominal_value=1  t_nominal_unit=N*m
      settings: InternalSimscapePortConfiguration="{\"Bottom\":[],\"Left\":[{\"id\":\"I\",\"label\":\"\",\"type\":\"foundation.mechanical.rotational.rotational\"}],\"Right\":[{\"id\":\"J\",\"label\":\"\",\"type\":\"foundation.mechanical.rotational.rotational\"}],\"Top\":[]}"
  Inertia Driveshaft FL : fl_lib/Mechanical/Rotational Elements/Inertia  inertia=HMPST.DriveshaftFL.J kg*m^2  num_ports=foundation.enum.numPorts2.two  w_specify=off  w_priority=High  w=0 rad/s  w_nominal_specify=off  w_nominal_value=1  w_nominal_unit=rad/s  t_specify=off  t_priority=None  t=0 N*m  t_nominal_specify=off  t_nominal_value=1  t_nominal_unit=N*m
      settings: InternalSimscapePortConfiguration="{\"Bottom\":[],\"Left\":[{\"id\":\"I\",\"label\":\"\",\"type\":\"foundation.mechanical.rotational.rotational\"}],\"Right\":[{\"id\":\"J\",\"label\":\"\",\"type\":\"foundation.mechanical.rotational.rotational\"}],\"Top\":[]}"
  Inertia Driveshaft FR : fl_lib/Mechanical/Rotational Elements/Inertia  inertia=HMPST.DriveshaftFR.J kg*m^2  num_ports=foundation.enum.numPorts2.two  w_specify=off  w_priority=High  w=0 rad/s  w_nominal_specify=off  w_nominal_value=1  w_nominal_unit=rad/s  t_specify=off  t_priority=None  t=0 N*m  t_nominal_specify=off  t_nominal_value=1  t_nominal_unit=N*m
      settings: InternalSimscapePortConfiguration="{\"Bottom\":[],\"Left\":[{\"id\":\"I\",\"label\":\"\",\"type\":\"foundation.mechanical.rotational.rotational\"}],\"Right\":[{\"id\":\"J\",\"label\":\"\",\"type\":\"foundation.mechanical.rotational.rotational\"}],\"Top\":[]}"
  Inertia Driveshaft RL : fl_lib/Mechanical/Rotational Elements/Inertia  inertia=HMPST.DriveshaftRL.J kg*m^2  num_ports=foundation.enum.numPorts2.two  w_specify=off  w_priority=High  w=0 rad/s  w_nominal_specify=off  w_nominal_value=1  w_nominal_unit=rad/s  t_specify=off  t_priority=None  t=0 N*m  t_nominal_specify=off  t_nominal_value=1  t_nominal_unit=N*m
      settings: InternalSimscapePortConfiguration="{\"Bottom\":[],\"Left\":[{\"id\":\"I\",\"label\":\"\",\"type\":\"foundation.mechanical.rotational.rotational\"}],\"Right\":[{\"id\":\"J\",\"label\":\"\",\"type\":\"foundation.mechanical.rotational.rotational\"}],\"Top\":[]}"
  Inertia Driveshaft RR : fl_lib/Mechanical/Rotational Elements/Inertia  inertia=HMPST.DriveshaftRR.J kg*m^2  num_ports=foundation.enum.numPorts2.two  w_specify=off  w_priority=High  w=0 rad/s  w_nominal_specify=off  w_nominal_value=1  w_nominal_unit=rad/s  t_specify=off  t_priority=None  t=0 N*m  t_nominal_specify=off  t_nominal_value=1  t_nominal_unit=N*m
      settings: InternalSimscapePortConfiguration="{\"Bottom\":[],\"Left\":[{\"id\":\"I\",\"label\":\"\",\"type\":\"foundation.mechanical.rotational.rotational\"}],\"Right\":[{\"id\":\"J\",\"label\":\"\",\"type\":\"foundation.mechanical.rotational.rotational\"}],\"Top\":[]}"
  Spring : fl_lib/Mechanical/Rotational Elements/Rotational Spring  spr_rate=HMPST.DriveshaftF.K N*m/rad  w_specify=off  w_priority=None  w=0 rad/s  w_nominal_specify=off  w_nominal_value=1  w_nominal_unit=rad/s  t_specify=off  t_priority=None  t=0 N*m  t_nominal_specify=off  t_nominal_value=1  t_nominal_unit=N*m  phi_specify=off  phi_priority=High  phi=0 rad  phi_nominal_specify=off  phi_nominal_value=1  phi_nominal_unit=rad
  RL : PMIOPort  Side=Left
  TransA : PMIOPort  Port=2  Side=Left
  FL : PMIOPort  Port=3  Side=Left
  RR : PMIOPort  Port=4  Side=Right
  Trans : PMIOPort  Port=5  Side=Right
  FR : PMIOPort  Port=6  Side=Right
  connections:
  Differential Rear/LConn1 -- Gear Output Transfer/RConn1 -- Inertia Driveshaft Rear/LConn1
  Inertia Carrier FR/LConn1 -- FR/RConn1
  Inertia Carrier FR/RConn1 -- Gear Sun FR/RConn1
  Differential Front/RConn1 -- Inertia Driveshaft FR/RConn1
  Inertia Driveshaft FR/LConn1 -- Gear Sun FR/LConn1
  Inertia Driveshaft FL/RConn1 -- Differential Front/RConn2
  Inertia Driveshaft FL/LConn1 -- Gear Sun LF/LConn1
  Inertia Carrier FL/RConn1 -- Gear Sun LF/RConn1
  Inertia Carrier FL/LConn1 -- FL/RConn1
  Inertia Carrier RR/LConn1 -- RR/RConn1
  Inertia Carrier RR/RConn1 -- Gear Sun RR/RConn1
  Inertia Driveshaft RR/RConn1 -- Differential Rear/RConn1
  Inertia Driveshaft RR/LConn1 -- Gear Sun RR/LConn1
  Inertia Driveshaft RL/RConn1 -- Differential Rear/RConn2
  Inertia Driveshaft RL/LConn1 -- Gear Sun LR/LConn1
  Inertia Carrier RL/RConn1 -- Gear Sun LR/RConn1
  Inertia Carrier RL/LConn1 -- RL/RConn1
  Damper/LConn1 -- Spring/LConn1 -- Differential Front/LConn1
  Gear Output Transfer/LConn1 -- TransA/RConn1 -- Trans/RConn1
  Damper/RConn1 -- Inertia Driveshaft Rear/RConn1 -- Spring/RConn1

== system sm_wheel_loader_lib/Wheel Loader Vehicle/Driveline/Driveline/Driveline 1D/Planetary FL ==
  note: Connections here for left side of vehicle.
      | Opposite from right side.
  Carrier : Subsystem  Tag=E5EDD8BF-BFC4-A349-9C21-406C76E99105
  Mechanical Rotational Reference : fl_lib/Mechanical/Rotational Elements/Mechanical Rotational Reference
  Revolute Ring Carrier : sm_lib/Joints/Revolute Joint  JointMode=Normal  CompositeWrenchDir=FollowerOnBase  CompositeWrenchFrame=BaseFrame  SenseConstraintForce=off  SenseConstraintTorque=off  SenseTotalForce=off  SenseTotalTorque=off  PositionTargetSpecify=off  PositionTargetPriority=High  PositionTargetValue=0  PositionTargetValueUnits=deg  VelocityTargetSpecify=off  VelocityTargetPriority=High  VelocityTargetValue=0  VelocityTargetValueUnits=deg/s  EquilibriumPosition=0  EquilibriumPositionUnits=deg  SpringStiffness=0  SpringStiffnessUnits=N*m/deg  DampingCoefficient=0  DampingCoefficientUnits=N*m/(deg/s)  LowerLimitSpecify=off  LowerLimitBound=-90  LowerLimitBoundUnits=deg  LowerLimitStiffness=1e4  LowerLimitStiffnessUnits=N*m/deg  LowerLimitDamping=10  LowerLimitDampingUnits=N*m/(deg/s)  LowerLimitTransitionRegionWidth=0.1  LowerLimitTransitionRegionWidthUnits=deg  UpperLimitSpecify=off  UpperLimitBound=90  UpperLimitBoundUnits=deg  UpperLimitStiffness=1e4  UpperLimitStiffnessUnits=N*m/deg  UpperLimitDamping=10  UpperLimitDampingUnits=N*m/(deg/s)  UpperLimitTransitionRegionWidth=0.1  UpperLimitTransitionRegionWidthUnits=deg  TorqueActuationMode=InputTorque  MotionActuationMode=ComputedMotion  SensePosition=off  SenseVelocity=on  SenseAcceleration=off  SenseTorqueForce=off  SenseLowerLimitTorqueForce=off  SenseUpperLimitTorqueForce=off
  Ring Gear : Subsystem  Tag=B2A6520B-B79A-3144-97C4-6FFE059DED13
  Rotational Multibody Interface : fl_lib/Mechanical/Multibody Interfaces/Rotational Multibody Interface
  R1 : PMIOPort  Side=Right
  "   C" : PMIOPort  Port=2  Side=Right
  C1 : PMIOPort  Port=3  Side=Left
  "   R" : PMIOPort  Port=4  Side=Right
  connections:
  C1/RConn1 -- Carrier/LConn1 -- Revolute Ring Carrier/RConn1
  Ring Gear/LConn1 -- Revolute Ring Carrier/LConn1 -- "   R"/RConn1 -- R1/RConn1
  Revolute Ring Carrier/RConn2 -- Rotational Multibody Interface/RConn1
  Rotational Multibody Interface/LConn1 -- Revolute Ring Carrier/LConn2
  Mechanical Rotational Reference/LConn1 -- Rotational Multibody Interface/LConn2
  "   C"/RConn1 -- Rotational Multibody Interface/RConn2

== system sm_wheel_loader_lib/Wheel Loader Vehicle/Driveline/Driveline/Driveline 1D/Planetary FR ==
  note: Connections here for right side of vehicle.
      | Opposite from left side.
  Carrier : Subsystem  Tag=E5EDD8BF-BFC4-A349-9C21-406C76E99105
  Mechanical Rotational Reference : fl_lib/Mechanical/Rotational Elements/Mechanical Rotational Reference
  Revolute Ring Carrier : sm_lib/Joints/Revolute Joint  JointMode=Normal  CompositeWrenchDir=FollowerOnBase  CompositeWrenchFrame=BaseFrame  SenseConstraintForce=off  SenseConstraintTorque=off  SenseTotalForce=off  SenseTotalTorque=off  PositionTargetSpecify=off  PositionTargetPriority=High  PositionTargetValue=0  PositionTargetValueUnits=deg  VelocityTargetSpecify=off  VelocityTargetPriority=High  VelocityTargetValue=0  VelocityTargetValueUnits=deg/s  EquilibriumPosition=0  EquilibriumPositionUnits=deg  SpringStiffness=0  SpringStiffnessUnits=N*m/deg  DampingCoefficient=0  DampingCoefficientUnits=N*m/(deg/s)  LowerLimitSpecify=off  LowerLimitBound=-90  LowerLimitBoundUnits=deg  LowerLimitStiffness=1e4  LowerLimitStiffnessUnits=N*m/deg  LowerLimitDamping=10  LowerLimitDampingUnits=N*m/(deg/s)  LowerLimitTransitionRegionWidth=0.1  LowerLimitTransitionRegionWidthUnits=deg  UpperLimitSpecify=off  UpperLimitBound=90  UpperLimitBoundUnits=deg  UpperLimitStiffness=1e4  UpperLimitStiffnessUnits=N*m/deg  UpperLimitDamping=10  UpperLimitDampingUnits=N*m/(deg/s)  UpperLimitTransitionRegionWidth=0.1  UpperLimitTransitionRegionWidthUnits=deg  TorqueActuationMode=InputTorque  MotionActuationMode=ComputedMotion  SensePosition=off  SenseVelocity=on  SenseAcceleration=off  SenseTorqueForce=off  SenseLowerLimitTorqueForce=off  SenseUpperLimitTorqueForce=off
  Ring Gear : Subsystem  Tag=B2A6520B-B79A-3144-97C4-6FFE059DED13
  Rotational Multibody Interface : fl_lib/Mechanical/Multibody Interfaces/Rotational Multibody Interface
  "   R" : PMIOPort  Side=Left
  "   C" : PMIOPort  Port=2  Side=Right
  C1 : PMIOPort  Port=3  Side=Left
  R1 : PMIOPort  Port=4  Side=Left
  connections:
  Revolute Ring Carrier/RConn1 -- Ring Gear/LConn1 -- R1/RConn1 -- "   R"/RConn1
  "   C"/RConn1 -- Revolute Ring Carrier/LConn1 -- Carrier/LConn1
  Rotational Multibody Interface/RConn1 -- Revolute Ring Carrier/RConn2
  Revolute Ring Carrier/LConn2 -- Rotational Multibody Interface/LConn1
  Mechanical Rotational Reference/LConn1 -- Rotational Multibody Interface/LConn2
  C1/RConn1 -- Rotational Multibody Interface/RConn2

== system sm_wheel_loader_lib/Wheel Loader Vehicle/Driveline/Driveline/Driveline 1D/Planetary RL ==
  note: Connections here for left side of vehicle.
      | Opposite from right side.
  Carrier : Subsystem  Tag=E5EDD8BF-BFC4-A349-9C21-406C76E99105
  Mechanical Rotational Reference : fl_lib/Mechanical/Rotational Elements/Mechanical Rotational Reference
  Revolute Ring Carrier : sm_lib/Joints/Revolute Joint  JointMode=Normal  CompositeWrenchDir=FollowerOnBase  CompositeWrenchFrame=BaseFrame  SenseConstraintForce=off  SenseConstraintTorque=off  SenseTotalForce=off  SenseTotalTorque=off  PositionTargetSpecify=off  PositionTargetPriority=High  PositionTargetValue=0  PositionTargetValueUnits=deg  VelocityTargetSpecify=off  VelocityTargetPriority=High  VelocityTargetValue=0  VelocityTargetValueUnits=deg/s  EquilibriumPosition=0  EquilibriumPositionUnits=deg  SpringStiffness=0  SpringStiffnessUnits=N*m/deg  DampingCoefficient=0  DampingCoefficientUnits=N*m/(deg/s)  LowerLimitSpecify=off  LowerLimitBound=-90  LowerLimitBoundUnits=deg  LowerLimitStiffness=1e4  LowerLimitStiffnessUnits=N*m/deg  LowerLimitDamping=10  LowerLimitDampingUnits=N*m/(deg/s)  LowerLimitTransitionRegionWidth=0.1  LowerLimitTransitionRegionWidthUnits=deg  UpperLimitSpecify=off  UpperLimitBound=90  UpperLimitBoundUnits=deg  UpperLimitStiffness=1e4  UpperLimitStiffnessUnits=N*m/deg  UpperLimitDamping=10  UpperLimitDampingUnits=N*m/(deg/s)  UpperLimitTransitionRegionWidth=0.1  UpperLimitTransitionRegionWidthUnits=deg  TorqueActuationMode=InputTorque  MotionActuationMode=ComputedMotion  SensePosition=off  SenseVelocity=on  SenseAcceleration=off  SenseTorqueForce=off  SenseLowerLimitTorqueForce=off  SenseUpperLimitTorqueForce=off
  Ring Gear : Subsystem  Tag=B2A6520B-B79A-3144-97C4-6FFE059DED13
  Rotational Multibody Interface : fl_lib/Mechanical/Multibody Interfaces/Rotational Multibody Interface
  "   R" : PMIOPort  Side=Right
  C1 : PMIOPort  Port=2  Side=Left
  "   C" : PMIOPort  Port=3  Side=Right
  R1 : PMIOPort  Port=4  Side=Right
  connections:
  Revolute Ring Carrier/LConn1 -- Ring Gear/LConn1 -- R1/RConn1 -- "   R"/RConn1
  Revolute Ring Carrier/RConn1 -- Carrier/LConn1 -- C1/RConn1
  Rotational Multibody Interface/RConn1 -- Revolute Ring Carrier/RConn2
  Revolute Ring Carrier/LConn2 -- Rotational Multibody Interface/LConn1
  Mechanical Rotational Reference/LConn1 -- Rotational Multibody Interface/LConn2
  "   C"/RConn1 -- Rotational Multibody Interface/RConn2

== system sm_wheel_loader_lib/Wheel Loader Vehicle/Driveline/Driveline/Driveline 1D/Planetary RR ==
  note: Connections here for right side of vehicle.
      | Opposite from left side.
  Carrier : Subsystem  Tag=E5EDD8BF-BFC4-A349-9C21-406C76E99105
  Mechanical Rotational Reference : fl_lib/Mechanical/Rotational Elements/Mechanical Rotational Reference
  Revolute Ring Carrier : sm_lib/Joints/Revolute Joint  JointMode=Normal  CompositeWrenchDir=FollowerOnBase  CompositeWrenchFrame=BaseFrame  SenseConstraintForce=off  SenseConstraintTorque=off  SenseTotalForce=off  SenseTotalTorque=off  PositionTargetSpecify=off  PositionTargetPriority=High  PositionTargetValue=0  PositionTargetValueUnits=deg  VelocityTargetSpecify=off  VelocityTargetPriority=High  VelocityTargetValue=0  VelocityTargetValueUnits=deg/s  EquilibriumPosition=0  EquilibriumPositionUnits=deg  SpringStiffness=0  SpringStiffnessUnits=N*m/deg  DampingCoefficient=0  DampingCoefficientUnits=N*m/(deg/s)  LowerLimitSpecify=off  LowerLimitBound=-90  LowerLimitBoundUnits=deg  LowerLimitStiffness=1e4  LowerLimitStiffnessUnits=N*m/deg  LowerLimitDamping=10  LowerLimitDampingUnits=N*m/(deg/s)  LowerLimitTransitionRegionWidth=0.1  LowerLimitTransitionRegionWidthUnits=deg  UpperLimitSpecify=off  UpperLimitBound=90  UpperLimitBoundUnits=deg  UpperLimitStiffness=1e4  UpperLimitStiffnessUnits=N*m/deg  UpperLimitDamping=10  UpperLimitDampingUnits=N*m/(deg/s)  UpperLimitTransitionRegionWidth=0.1  UpperLimitTransitionRegionWidthUnits=deg  TorqueActuationMode=InputTorque  MotionActuationMode=ComputedMotion  SensePosition=off  SenseVelocity=on  SenseAcceleration=off  SenseTorqueForce=off  SenseLowerLimitTorqueForce=off  SenseUpperLimitTorqueForce=off
  Ring Gear : Subsystem  Tag=B2A6520B-B79A-3144-97C4-6FFE059DED13
  Rotational Multibody Interface : fl_lib/Mechanical/Multibody Interfaces/Rotational Multibody Interface
  R1 : PMIOPort  Side=Left
  C1 : PMIOPort  Port=2  Side=Left
  "   C" : PMIOPort  Port=3  Side=Right
  "   R" : PMIOPort  Port=4  Side=Left
  connections:
  Revolute Ring Carrier/LConn1 -- "   C"/RConn1 -- Carrier/LConn1
  Ring Gear/LConn1 -- "   R"/RConn1 -- R1/RConn1 -- Revolute Ring Carrier/RConn1
  Rotational Multibody Interface/RConn1 -- Revolute Ring Carrier/RConn2
  Revolute Ring Carrier/LConn2 -- Rotational Multibody Interface/LConn1
  Mechanical Rotational Reference/LConn1 -- Rotational Multibody Interface/LConn2
  C1/RConn1 -- Rotational Multibody Interface/RConn2

== system sm_wheel_loader_lib/Wheel Loader Vehicle/Driveline/Driveline/Driveline 3D/Center Shaft ==
  Center Bearing : Subsystem  Tag=B404EA4B-CCBB-5D4C-9E00-516187D4968A
  Shaft Midship : Subsystem  Tag=1CA4EEB4-9711-B949-9B74-FDF79E4E06F5
  B2 : PMIOPort  Side=Left
  B1 : PMIOPort  Port=2  Side=Right
  connections:
  B2/RConn1 -- Center Bearing/RConn1
  Center Bearing/LConn1 -- Shaft Midship/RConn1
  B1/RConn1 -- Shaft Midship/LConn1
